simulink library "Pitch_Actuation_Lib"  (R2025a)
settings: Solver=ode45  StartTime=0.0  StopTime=10.0  RelTol=1e-3  EnableMultiTasking=on
undefined symbols (not defined in the file or in its folder): Actuator_Lookup, WT_Params
libraries: Hydraulic_Actuator_Lib x3
Description:
  | Copyright 2009-2025 The MathWorks, Inc. MathWorks, Inc.
settings Model: Creator=smiller  LastModifiedBy=smiller
settings SolverCC: AlgebraicLoopSolver=TrustRegion
settings DataIOCC: LimitDataPoints=on  SaveFormat=Array  SignalLoggingSaveFormat=ModelDataLogs  ReturnWorkspaceOutputs=off
settings OptimizationCC: ReuseModelBlockBuffer=off  ExpressionDepthLimit=2147483647.0  LifeSpan=inf
settings DebuggingCC: UnderspecifiedInitializationDetection=Classic  MergeDetectMultiDrivingBlocksExec=none  SolverPrmCheckMsg=warning  FcnCallInpInsideContextMsg=warning  UnconnectedInputMsg=warning  UnconnectedOutputMsg=warning  UnconnectedLineMsg=warning  AllowSymbolicDim=off  StateNameClashWarn=warning  PregeneratedLibrarySubsystemCodeDiagnostic=none  SFUnexpectedBacktrackingDiag=warning  SFNoUnconditionalDefaultTransitionDiag=warning  SFExecutionAtInitializationDiag=none  ArithmeticOperatorsInVariantConditions=warning
settings HardwareCC: ProdBitPerPointer=32.0  ProdBitPerSizeT=32.0  ProdBitPerPtrDiffT=32.0  ProdLargestAtomicFloat=None  ProdIntDivRoundTo=Undefined  ProdEndianess=Unspecified  ProdWordSize=32.0  ProdHWDeviceType=32-bit Generic
settings ModelReferenceCC: EnableRefExpFcnMdlSchedulingChecks=on  PropagateSignalLabelsOutOfModel=off
settings SFSimCC: SimUseLocalCustomCode=off  CustomCodeUndefinedFunction=UseInterfaceOnly
settings RTWCC: RTWUseLocalCustomCode=off  GPUComputeCapability=3.5  DLArmComputeVersion=19.05
settings CodeAppCC: StateflowObjectComments=on
settings GRTTargetCC: TargetLangStandard=C89/C90 (ANSI)  CombineOutputUpdateFcns=off  GRTInterface=on
settings ConfigComp: CovMetricSettings=dw  CovSaveCumulativeToWorkspaceVar=on  CovSaveSingleToWorkspaceVar=on  CovExternalEMLEnable=off  CovSFcnEnable=off

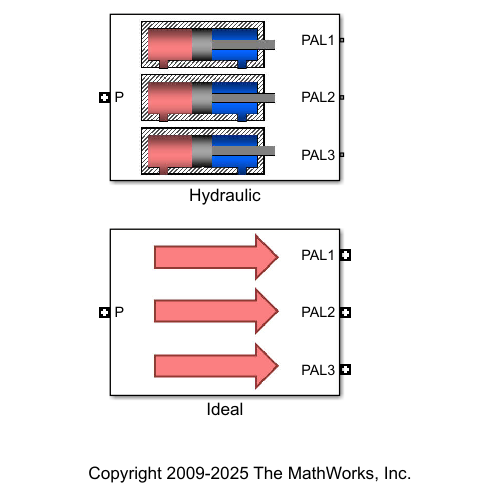
[thumbnail: Simulink's stored preview of the top-level diagram]
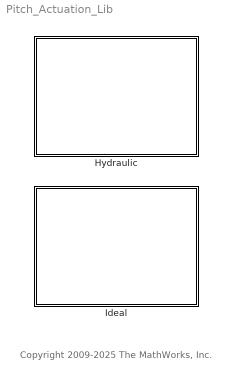
== system Pitch_Actuation_Lib ==
  note: Copyright 2009-2025 The MathWorks, Inc.
  Hydraulic : Subsystem
      mask Display: image('Pitch_Hydraulic_Actuation_IMAGE.jpg');
  Ideal : Subsystem
      mask Display: image('Pitch_Ideal_Actuation_IMAGE.jpg');

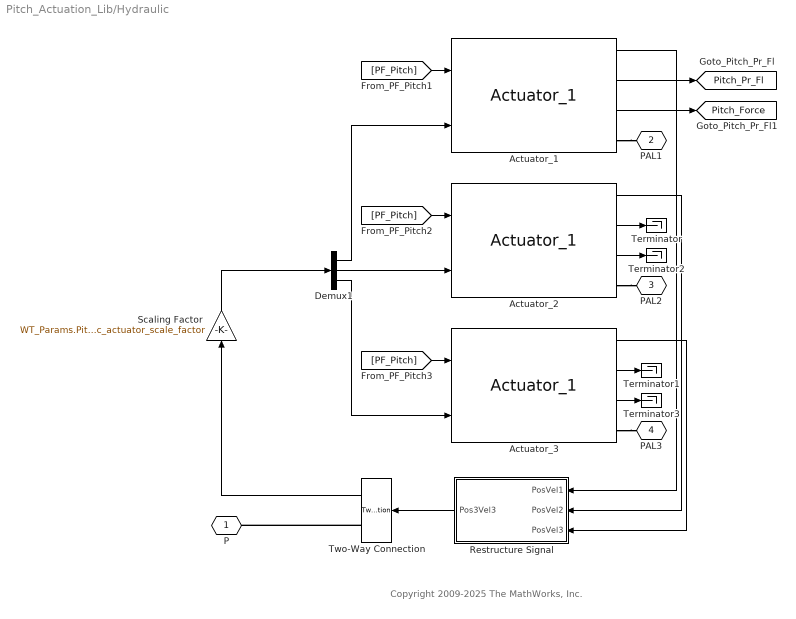
== system Pitch_Actuation_Lib/Hydraulic ==
  note: Copyright 2009-2025 The MathWorks, Inc.
  Actuator_1 : Hydraulic_Actuator_Lib/Actuator_1  SystemSampleTime=-1  VariantActivationTime=update diagram  EmptyChoice=off  PassThrough=off  PassThroughVariantControl=(default)  EmptyChoiceVariantControl=(default)  AllowFlexibleInterface=on  Latency=0  AutoFrameSizeCalculation=off
  Actuator_2 : Hydraulic_Actuator_Lib/Actuator_1  SystemSampleTime=-1  VariantActivationTime=update diagram  EmptyChoice=off  PassThrough=off  PassThroughVariantControl=(default)  EmptyChoiceVariantControl=(default)  AllowFlexibleInterface=on  Latency=0  AutoFrameSizeCalculation=off
  Actuator_3 : Hydraulic_Actuator_Lib/Actuator_1  SystemSampleTime=-1  VariantActivationTime=update diagram  EmptyChoice=off  PassThrough=off  PassThroughVariantControl=(default)  EmptyChoiceVariantControl=(default)  AllowFlexibleInterface=on  Latency=0  AutoFrameSizeCalculation=off
  Demux1 : Demux  Outputs=3
  Restructure Signal : Subsystem
  Scaling Factor : Gain  Gain=WT_Params.Pitch_Actuator.hydraulic_actuator_scale_factor
  Terminator{,1..3} (4 alike) : Terminator
  Two-Way Connection : TwoWayConnection
  P : PMIOPort  Tag=PMCPort  Side=Left
  PAL1 : PMIOPort  Tag=PMCPort  Port=2  Side=Right
  PAL2 : PMIOPort  Tag=PMCPort  Port=3  Side=Right
  PAL3 : PMIOPort  Tag=PMCPort  Port=4  Side=Right
  tag scope: Pitch_Force=global, Pitch_Pr_Fl=global
  wires:
  Actuator_1/2 -> [Pitch_Pr_Fl]
  Restructure Signal/1(Pos3Vel3) -> Two-Way Connection/1
  Actuator_1/1 -> Restructure Signal/1(PosVel1)
  Actuator_2/1 -> Restructure Signal/2(PosVel2)
  Actuator_3/1 -> Restructure Signal/3(PosVel3)
  Two-Way Connection/1 -> Scaling Factor/1
  [PF_Pitch] -> Actuator_1/1
  [PF_Pitch] -> Actuator_2/1
  [PF_Pitch] -> Actuator_3/1
  Demux1/1 -> Actuator_1/2
  Demux1/2 -> Actuator_2/2
  Demux1/3 -> Actuator_3/2
  Actuator_2/2 -> Terminator/1
  Actuator_3/2 -> Terminator1/1
  Scaling Factor/1 -> Demux1/1
  Actuator_2/3 -> Terminator2/1
  Actuator_3/3 -> Terminator3/1
  Actuator_1/3 -> [Pitch_Force]
  connections:
  Two-Way Connection/RConn1 -- P/RConn1
  Actuator_1/RConn1 -- PAL1/RConn1
  Actuator_2/RConn1 -- PAL2/RConn1
  Actuator_3/RConn1 -- PAL3/RConn1

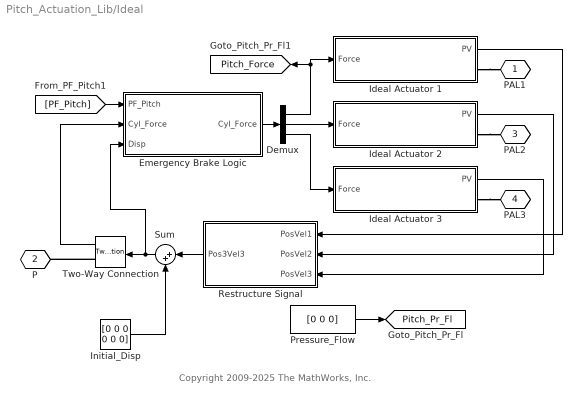
== system Pitch_Actuation_Lib/Ideal ==
  note: Copyright 2009-2025 The MathWorks, Inc.
  Demux : Demux  Outputs=3
  Emergency Brake Logic : Subsystem
  Ideal Actuator 1 : Subsystem
      mask Display: image(imread('Pitch_Ideal_Actuator_IMAGE.jpg'));
  Ideal Actuator 2 : Subsystem
      mask Display: image(imread('Pitch_Ideal_Actuator_IMAGE.jpg'));
  Ideal Actuator 3 : Subsystem
      mask Display: image(imread('Pitch_Ideal_Actuator_IMAGE.jpg'));
  Initial_Disp : Constant  Value=[0 0 0 0 0 0]
  Pressure_Flow : Constant  Value=[0 0 0]
  Restructure Signal : Subsystem
  Sum : Sum  Inputs=|++
  Two-Way Connection : TwoWayConnection
  PAL1 : PMIOPort  Tag=PMCPort  Side=Right
  P : PMIOPort  Tag=PMCPort  Port=2  Side=Left
  PAL2 : PMIOPort  Tag=PMCPort  Port=3  Side=Right
  PAL3 : PMIOPort  Tag=PMCPort  Port=4  Side=Right
  tag scope: Pitch_Force=global, Pitch_Pr_Fl=global
  wires:
  Pressure_Flow/1 -> [Pitch_Pr_Fl]
  Demux/3 -> Ideal Actuator 3/1(Force)
  Demux/2 -> Ideal Actuator 2/1(Force)
  Demux/1 -> Ideal Actuator 1/1(Force), [Pitch_Force]
  Emergency Brake Logic/1(Cyl_Force) -> Demux/1
  [PF_Pitch] -> Emergency Brake Logic/1(PF_Pitch)
  Ideal Actuator 3/1(PV) -> Restructure Signal/3(PosVel3)
  Ideal Actuator 2/1(PV) -> Restructure Signal/2(PosVel2)
  Two-Way Connection/1 -> Emergency Brake Logic/2("Cyl_Force ")
  Initial_Disp/1 -> Sum/2
  Sum/1 -> Two-Way Connection/1, Emergency Brake Logic/3(Disp)
  Restructure Signal/1(Pos3Vel3) -> Sum/1
  Ideal Actuator 1/1(PV) -> Restructure Signal/1(PosVel1)
  connections:
  Two-Way Connection/RConn1 -- P/RConn1
  Ideal Actuator 1/RConn1 -- PAL1/RConn1
  Ideal Actuator 2/RConn1 -- PAL2/RConn1
  Ideal Actuator 3/RConn1 -- PAL3/RConn1

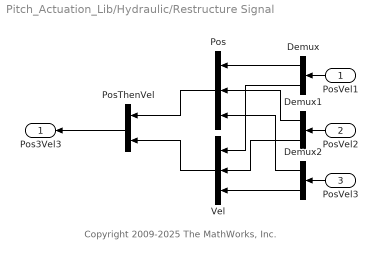
== system Pitch_Actuation_Lib/Hydraulic/Restructure Signal ==
  note: Copyright 2009-2025 The MathWorks, Inc.
  PosVel1 : Inport
  PosVel2 : Inport  Port=2
  PosVel3 : Inport  Port=3
  Demux : Demux  Outputs=2
  Demux1 : Demux  Outputs=2
  Demux2 : Demux  Outputs=2
  Pos : Mux  Inputs=3
  PosThenVel : Mux  Inputs=2
  Vel : Mux  Inputs=3
  Pos3Vel3 : Outport  VectorParamsAs1DForOutWhenUnconnected=off
  wires:
  Vel/1 -> PosThenVel/2
  Pos/1 -> PosThenVel/1
  Demux2/2 -> Vel/3
  Demux1/2 -> Vel/2
  Demux/2 -> Vel/1
  Demux2/1 -> Pos/3
  Demux1/1 -> Pos/2
  Demux/1 -> Pos/1
  PosVel3/1 -> Demux2/1
  PosVel2/1 -> Demux1/1
  PosVel1/1 -> Demux/1
  PosThenVel/1 -> Pos3Vel3/1

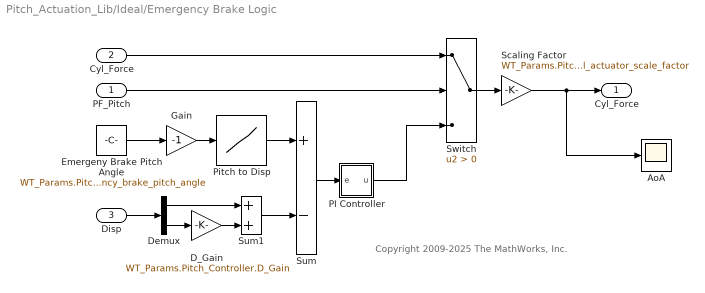
== system Pitch_Actuation_Lib/Ideal/Emergency Brake Logic ==
  note: Copyright 2009-2025 The MathWorks, Inc.
  PF_Pitch : Inport
  "Cyl_Force " : Inport  Port=2
  Disp : Inport  Port=3
  AoA : Scope
      settings: TimeSpan=600  ActiveDisplayYMinimum=0  ActiveDisplayYMaximum=100  DataLoggingVariableName=ScopeData10
  D_Gain : Gain  Gain=WT_Params.Pitch_Controller.D_Gain
  Demux : Demux  Outputs=2
  Emergeny Brake Pitch Angle : Constant  Value=WT_Params.Pitch_Controller.emergency_brake_pitch_angle
  Gain : Gain  Gain=-1
  PI Controller : Subsystem  mask(PID Controller){P=WT_Params.Pitch_Controller.P_Gain, I=WT_Params.Pitch_Controller.I_Gain}
      mask prompts: P "Proportional:"; I "Integral:"
      mask help:
      | Enter expressions for proportional, integral, and derivative terms.
      | P+I/s+Ds
      mask Help: This block implements a PID controller where parameters are entered for the Proportional, Integral and Derivative terms. Unmask this block to see how it works. The derivative term is implemented using a true derivative block.
      mask Display: disp('PI')
  Pitch to Disp : Lookup  InputValues=-Actuator_Lookup.angle  Table=Actuator_Lookup.extension  SaturateOnIntegerOverflow=off
  Scaling Factor : Gain  Gain=WT_Params.Pitch_Actuator.ideal_actuator_scale_factor
  Sum : Sum  Inputs=+-
  Sum1 : Sum
  Switch : Switch  Criteria=u2 > Threshold  SaturateOnIntegerOverflow=off  InputSameDT=off
  Cyl_Force : Outport  VectorParamsAs1DForOutWhenUnconnected=off
  wires:
  Gain/1 -> Pitch to Disp/1
  Switch/1 -> Scaling Factor/1
  PF_Pitch/1 -> Switch/2
  "Cyl_Force "/1 -> Switch/1
  Emergeny Brake Pitch Angle/1 -> Gain/1
  Disp/1 -> Demux/1
  Sum/1 -> PI Controller/1(e)
  Pitch to Disp/1 -> Sum/1
  Sum1/1 -> Sum/2
  Demux/1 -> Sum1/1
  Demux/2 -> D_Gain/1
  D_Gain/1 -> Sum1/2
  PI Controller/1(u) -> Switch/3
  Scaling Factor/1 -> Cyl_Force/1, AoA/1

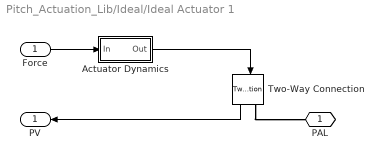
== system Pitch_Actuation_Lib/Ideal/Ideal Actuator 1 ==
  Force : Inport
  Actuator Dynamics : Subsystem  mask(First-order lag supporting vector signals){b=WT_Params.Pitch_Actuator.ideal_actuator_time_constant, x_initial=0}
      mask prompts: b "Filter time constant"; x_initial "Initial output"
      mask help: Models a lag of the form 1/(b*s+1) where s is the Laplace operator.
  Two-Way Connection : TwoWayConnection
  PAL : PMIOPort  Side=Right
  PV : Outport  VectorParamsAs1DForOutWhenUnconnected=off
  wires:
  Two-Way Connection/1 -> PV/1
  Force/1 -> Actuator Dynamics/1(In)
  Actuator Dynamics/1(Out) -> Two-Way Connection/1
  connections:
  Two-Way Connection/RConn1 -- PAL/RConn1

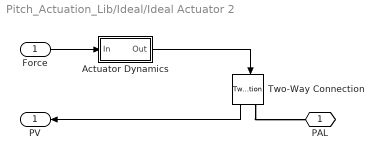
== system Pitch_Actuation_Lib/Ideal/Ideal Actuator 2 ==
  Force : Inport
  Actuator Dynamics : Subsystem  mask(First-order lag supporting vector signals){b=WT_Params.Pitch_Actuator.ideal_actuator_time_constant, x_initial=0}
      mask prompts: b "Filter time constant"; x_initial "Initial output"
      mask help: Models a lag of the form 1/(b*s+1) where s is the Laplace operator.
  Two-Way Connection : TwoWayConnection
  PAL : PMIOPort  Side=Right
  PV : Outport  VectorParamsAs1DForOutWhenUnconnected=off
  wires:
  Actuator Dynamics/1(Out) -> Two-Way Connection/1
  Force/1 -> Actuator Dynamics/1(In)
  Two-Way Connection/1 -> PV/1
  connections:
  Two-Way Connection/RConn1 -- PAL/RConn1

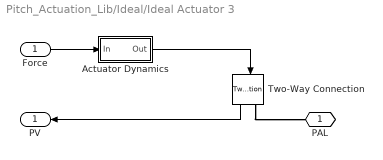
== system Pitch_Actuation_Lib/Ideal/Ideal Actuator 3 ==
  Force : Inport
  Actuator Dynamics : Subsystem  mask(First-order lag supporting vector signals){b=WT_Params.Pitch_Actuator.ideal_actuator_time_constant, x_initial=0}
      mask prompts: b "Filter time constant"; x_initial "Initial output"
      mask help: Models a lag of the form 1/(b*s+1) where s is the Laplace operator.
  Two-Way Connection : TwoWayConnection
  PAL : PMIOPort  Side=Right
  PV : Outport  VectorParamsAs1DForOutWhenUnconnected=off
  wires:
  Two-Way Connection/1 -> PV/1
  Force/1 -> Actuator Dynamics/1(In)
  Actuator Dynamics/1(Out) -> Two-Way Connection/1
  connections:
  Two-Way Connection/RConn1 -- PAL/RConn1

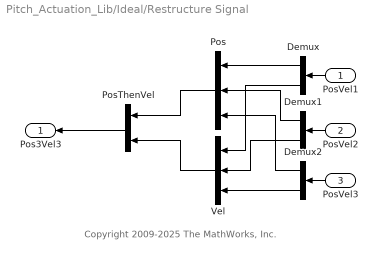
== system Pitch_Actuation_Lib/Ideal/Restructure Signal ==
  note: Copyright 2009-2025 The MathWorks, Inc.
  PosVel1 : Inport
  PosVel2 : Inport  Port=2
  PosVel3 : Inport  Port=3
  Demux : Demux  Outputs=2
  Demux1 : Demux  Outputs=2
  Demux2 : Demux  Outputs=2
  Pos : Mux  Inputs=3
  PosThenVel : Mux  Inputs=2
  Vel : Mux  Inputs=3
  Pos3Vel3 : Outport  VectorParamsAs1DForOutWhenUnconnected=off
  wires:
  PosThenVel/1 -> Pos3Vel3/1
  PosVel1/1 -> Demux/1
  PosVel2/1 -> Demux1/1
  PosVel3/1 -> Demux2/1
  Demux/1 -> Pos/1
  Demux1/1 -> Pos/2
  Demux2/1 -> Pos/3
  Demux/2 -> Vel/1
  Demux1/2 -> Vel/2
  Demux2/2 -> Vel/3
  Pos/1 -> PosThenVel/1
  Vel/1 -> PosThenVel/2

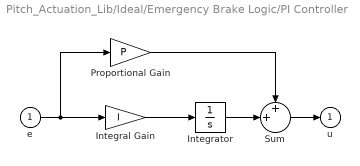
== system Pitch_Actuation_Lib/Ideal/Emergency Brake Logic/PI Controller ==
  e : Inport
  Integral Gain : Gain  Gain=I  SaturateOnIntegerOverflow=on  OutDataTypeStr=Inherit: Same as input  ParamDataTypeStr=Inherit: Same as input
  Integrator : Integrator
  Proportional Gain : Gain  Gain=P  SaturateOnIntegerOverflow=on  OutDataTypeStr=Inherit: Same as input  ParamDataTypeStr=Inherit: Same as input
  Sum : Sum  Inputs=++|  InputSameDT=on  SaturateOnIntegerOverflow=on  OutDataTypeStr=Inherit: Same as first input
  u : Outport  InitialOutput=0  VectorParamsAs1DForOutWhenUnconnected=off
  wires:
  Sum/1 -> u/1
  e/1 -> Integral Gain/1, Proportional Gain/1
  Integrator/1 -> Sum/2
  Proportional Gain/1 -> Sum/1
  Integral Gain/1 -> Integrator/1

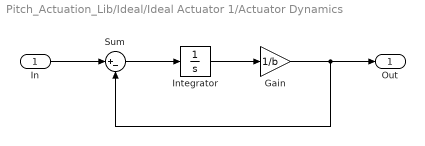
== system Pitch_Actuation_Lib/Ideal/Ideal Actuator 1/Actuator Dynamics ==
  In : Inport
  Gain : Gain  Gain=1/b
  Integrator : Integrator  InitialCondition=x_initial
  Sum : Sum  Inputs=|+-  InputSameDT=on  SaturateOnIntegerOverflow=on  OutDataTypeStr=Inherit: Same as first input
  Out : Outport  VectorParamsAs1DForOutWhenUnconnected=off
  wires:
  Sum/1 -> Integrator/1
  In/1 -> Sum/1
  Integrator/1 -> Gain/1
  Gain/1 -> Sum/2, Out/1

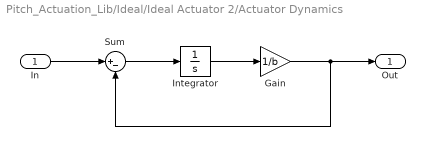
== system Pitch_Actuation_Lib/Ideal/Ideal Actuator 2/Actuator Dynamics ==
  In : Inport
  Gain : Gain  Gain=1/b
  Integrator : Integrator  InitialCondition=x_initial
  Sum : Sum  Inputs=|+-  InputSameDT=on  SaturateOnIntegerOverflow=on  OutDataTypeStr=Inherit: Same as first input
  Out : Outport  VectorParamsAs1DForOutWhenUnconnected=off
  wires:
  Gain/1 -> Out/1, Sum/2
  Integrator/1 -> Gain/1
  In/1 -> Sum/1
  Sum/1 -> Integrator/1

== system Pitch_Actuation_Lib/Ideal/Ideal Actuator 3/Actuator Dynamics ==
  In : Inport
  Gain : Gain  Gain=1/b
  Integrator : Integrator  InitialCondition=x_initial
  Sum : Sum  Inputs=|+-  InputSameDT=on  SaturateOnIntegerOverflow=on  OutDataTypeStr=Inherit: Same as first input
  Out : Outport  VectorParamsAs1DForOutWhenUnconnected=off
  wires:
  Sum/1 -> Integrator/1
  In/1 -> Sum/1
  Integrator/1 -> Gain/1
  Gain/1 -> Sum/2, Out/1
